simulink model "StampFly_StudentBlocks"  (R2026b)
settings: Solver=VariableStepAuto
undefined symbols (not defined in the file): Bottom, Official
(part 5 of 6)

== stateflow chart StampFly_StudentBlocks/Estimation/ToFHoldOutlierFilter ==
  note: ToF処理：新データ時に距離を更新。20 mm以下は保持、500 mmを超える飛びは最大2回補外。5 msフィルター。
  state Calculate
    en: [alt,raw]=stepFn(mm,fresh,mode,dt);
    du: [alt,raw]=stepFn(mm,fresh,mode,dt);
  (default) -> Calculate
  data: mm function_input; fresh function_input; mode function_input; dt function_input; alt function_output; raw function_output; mm input int16; fresh input uint8; mode input uint8; dt input single; alt output single; raw output int16
  function [alt,raw]=stepFn(mm,fresh,mode,dt):
    | function [alt,raw]=stepFn(mm,fresh,mode,dt)
    | % 日本語の説明はブロック注釈とDescriptionを参照。
    | %#codegen
    | persistent History Range Raw Outlier Alt PreviousMode;
    | if isempty(History)
    | History=zeros(4,1,'int16');
    | Range=int16(0);
    | Raw=int16(0);
    | Outlier=uint8(0);
    | Alt=single(0);
    | PreviousMode=uint8(0);
    | end
    |             if mode==3 && mode~=PreviousMode,History(:)=int16(0);Alt=single(0);end
    |             if mode>1
    |                 if fresh~=0
    |                     Raw=mm;if mm>int16(20),Range=mm;end
    |                     delta=int32(Range)-int32(History(2));
    |                     if abs(delta)>int32(500) && Outlier<uint8(2)
    |                         extrap=int32(History(2))+idivide(int32(History(2))-int32(History(4)),int32(2),'fix');
    |                         Range=int16(extrap);Outlier=Outlier+uint8(1);
    |                     else
    |                         Outlier=uint8(0);History(4)=History(3);History(3)=History(2);History(2)=Range;
    |                     end
    |                 end
    |                 Alt=filterStep(single(double(Range)/1000),dt,single(0.005),Alt);
    |             end
    |             alt=Alt;raw=Raw;PreviousMode=mode;
    | end
    | 
    | function s = filterStep(u,h,T,s)
    | %FILTERSTEP Exact Filter::update, including operation ordering.
    | %#codegen
    | s = s*T/(T+h) + u*h/(T+h);
    | end

== stateflow chart StampFly_StudentBlocks/LoggingAndStatus/StatusOutputs400/StatusIndicators400 ==
  note: LED・ブザー：校正、待機、飛行、低電圧、通信異常とモード変更を表示。色・周波数・再起動判定はモデル内。ハードウェアブロックは受け取った値だけを出力。
  state Calculate
    en: [color1,color2,tone,restart]=stepFn(mode,controlMode,altFlag,flipFlag,lowVoltage,rcError,ahrsFlag,button);
    du: [color1,color2,tone,restart]=stepFn(mode,controlMode,altFlag,flipFlag,lowVoltage,rcError,ahrsFlag,button);
  (default) -> Calculate
  data: arg_mode function_input; arg_controlMode function_input; arg_altFlag function_input; arg_flipFlag function_input; arg_lowVoltage function_input; arg_rcError function_input; arg_ahrsFlag function_input; arg_button function_input; arg_color1 function_output; arg_color2 function_output; arg_tone function_output; arg_restart function_output; mode input uint8; controlMode input single; altFlag input uint8; flipFlag input uint8; lowVoltage input uint8; rcError input uint8; ahrsFlag input uint8; button input uint8; color1 output uint32; color2 output uint32; tone output uint32; restart output boolean
  function [arg_color1,arg_color2,arg_tone,arg_restart]=stepFn(arg_mode,arg_controlMode,arg_altFlag,arg_flipFlag,arg_lowVoltage,arg_rcError,arg_ahrsFlag,arg_button):
    | function [arg_color1,arg_color2,arg_tone,arg_restart]=stepFn(arg_mode,arg_controlMode,arg_altFlag,arg_flipFlag,arg_lowVoltage,arg_rcError,arg_ahrsFlag,arg_button)
    | % 公式led_driveの状態色。ブザーの200ms待機は400Hzカウンターへ置換。
    | %#codegen
    | persistent Blink Rainbow C1 C2 Tick AHRSPrev ToneTicks ButtonCount WasPressed;
    | if isempty(Blink)
    |  Blink=uint16(0);Rainbow=uint32(255);C1=uint32(0);C2=uint32(0);Tick=uint16(0);AHRSPrev=uint8(0);ToneTicks=uint16(0);ButtonCount=uint8(0);WasPressed=false;
    | end
    | if arg_mode==1,C1=uint32(hex2dec('FF00FF'));C2=C1;
    | elseif arg_mode==5,C1=uint32(hex2dec('00FF00'));C2=C1;
    | elseif arg_mode==2
    |  c=uint32(hex2dec('FFFF00'));
    |  if arg_controlMode~=0,c=uint32(hex2dec('DC669B'));elseif arg_flipFlag~=0,c=uint32(hex2dec('FF9933'));end
    |  if arg_altFlag>=1,c=uint32(hex2dec('331155'));end
    |  if arg_rcError==1,c=uint32(hex2dec('FF0000'));end
    |  C1=c;C2=c;if arg_lowVoltage>=100,C1=uint32(hex2dec('18EBF9'));end
    | elseif arg_mode==3
    |  if arg_lowVoltage<100
    |   if Blink==0
    |    top=bitand(Rainbow,uint32(hex2dec('800000')))~=0;Rainbow=bitshift(Rainbow,1);if top,Rainbow=bitor(Rainbow,uint32(1));end
    |    C1=Rainbow;C2=Rainbow;Blink=Blink+uint16(1);
    |   end
    |   Blink=Blink+uint16(1);if Blink>20,Blink=uint16(0);end
    |  else
    |   if Blink<10,C1=uint32(hex2dec('18EBF9'));C2=C1;
    |   elseif Blink<200,C1=uint32(0);C2=uint32(0);else,Blink=uint16(0);end
    |   Blink=Blink+uint16(1);
    |  end
    |  if arg_ahrsFlag~=AHRSPrev && arg_ahrsFlag==1,ToneTicks=uint16(80);end
    |  AHRSPrev=arg_ahrsFlag;
    | end
    | arg_tone=uint32(0);
    | % Startup notes from official buzzer.h. Four 200ms notes, then silence.
    | if Tick<320
    |  notes=uint32([294 441 350 393]);idx=min(floor(double(Tick)/80)+1,4);arg_tone=notes(idx);Tick=Tick+uint16(1);
    | elseif ToneTicks>0,arg_tone=uint32(4000);ToneTicks=ToneTicks-uint16(1);end
    | arg_restart=false;
    | if arg_button==1,ButtonCount=min(ButtonCount+uint8(1),uint8(40));if ButtonCount>=4,WasPressed=true;end
    | elseif WasPressed,arg_restart=true;WasPressed=false;ButtonCount=uint8(0);else,ButtonCount=uint8(0);end
    | % FastLED brightness15, show32: cap displayed channels without changing logic.
    | arg_color1=scale(C1);arg_color2=scale(C2);
    | end
    | function c=scale(x)
    | r=bitand(bitshift(x,-16),uint32(255));g=bitand(bitshift(x,-8),uint32(255));b=bitand(x,uint32(255));
    | c=bitor(bitor(bitshift(uint32(double(r)*15/255),16),bitshift(uint32(double(g)*15/255),8)),uint32(double(b)*15/255));
    | end

== stateflow chart StampFly_StudentBlocks/Estimation/AltitudeKalman ==
  note: 高度Kalman：状態=[鉛直速度;高度;加速度バイアス]。400 Hzで最新保持ToFと鉛直加速度を使用。公式resetは内部推定xを保持。
  state Calculate
    en: [height,velocity,bias]=stepFn(alt,az,mode,dt,parkingReset);
    du: [height,velocity,bias]=stepFn(alt,az,mode,dt,parkingReset);
  (default) -> Calculate
  data: alt function_input; az function_input; mode function_input; dt function_input; parkingReset function_input; height function_output; velocity function_output; bias function_output; alt input single; az input single; mode input uint8; dt input single; parkingReset input boolean; height output single; velocity output single; bias output single
  function [height,velocity,bias]=stepFn(alt,az,mode,dt,parkingReset):
    | function [height,velocity,bias]=stepFn(alt,az,mode,dt,parkingReset)
    | % 日本語の説明はブロック注釈とDescriptionを参照。
    | %#codegen
    | persistent State First PreviousMode;
    | if isempty(State)
    | State=kalmanInitial();
    | First=false;
    | PreviousMode=uint8(0);
    | end
    |             if parkingReset,[~,State]=kalmanStep(single(0),single(0),dt,true,State);end
    |             if mode==3 && mode~=PreviousMode,First=false;end
    |             if mode>1
    |                 if First,[~,State]=kalmanStep(alt,az,dt,false,State);else,First=true;end
    |             end
    |             velocity=State.output(1);height=State.output(2);bias=State.output(3);PreviousMode=mode;
    | end
    | 
    | function [y,s] = kalmanStep(z,acc,h,resetState,s)
    | %KALMANSTEP Direct translation of Alt_kalman::update, state [v;z;bias].
    | % Preserve reset(): covariance and public output reset, private x is retained.
    | %#codegen
    | if resetState
    |     s.P = single(100)*eye(3,'single'); s.output(:) = single(0);
    | else
    |     p=s.P; b=single(-0.01); f=single(1)+h*b;
    |     xp=[s.x(1)+(acc-s.x(3))*h;s.x(2)+s.x(1)*h;s.x(3)*f];
    |     pp=zeros(3,3,'single');
    |     pp(1,1)=p(1,1)-h*(p(3,1)+p(1,3))+h*h*p(3,3)+h*h*single(0.01);
    |     pp(1,2)=h*(p(1,1)-p(3,2))-h*h*p(3,1)+p(1,2);
    |     pp(1,3)=f*(p(1,3)-h*p(3,3));
    |     pp(2,1)=h*(p(1,1)-p(2,3))-h*h*p(1,3)+p(2,1);
    |     pp(2,2)=h*h*p(1,1)+h*(p(2,1)+p(1,2))+p(2,2);
    |     pp(2,3)=f*(p(2,3)+h*p(1,3));
    |     pp(3,1)=f*(p(3,1)-h*p(3,3));
    |     pp(3,2)=f*(p(3,2)+h*p(3,1));
    |     pp(3,3)=f*f*p(3,3)+h*h;
    |     k=[pp(1,2);pp(2,2);pp(3,2)]/(pp(2,2)+single(0.004*0.004));
    |     e=z-xp(2); s.x=xp+k*e; s.output=s.x;
    |     s.P(1,:)=pp(1,:)-k(1)*pp(2,:);
    |     s.P(2,:)=pp(2,:)*(single(1)-k(2));
    |     s.P(3,:)=-k(3)*pp(2,:)+pp(3,:);
    | end
    | y=s.output;
    | end
    | 
    | function s = kalmanInitial()
    | %#codegen
    | s = struct('x',zeros(3,1,'single'),'P',single(100)*eye(3,'single'), ...
    |     'output',zeros(3,1,'single'));
    | end

== stateflow chart StampFly_StudentBlocks/Estimation/SensorFlags ==
  note: フラグ判定：OverG、距離無効/高度上限、低電圧100回。PID制御や状態遷移で使います。
  state Calculate
    en: [flags]=stepFn(accel,azd,voltage,mode,altFlag,height,rawRange,dt,parkingReset,flipFlag);
    du: [flags]=stepFn(accel,azd,voltage,mode,altFlag,height,rawRange,dt,parkingReset,flipFlag);
  (default) -> Calculate
  data: arg_accel function_input; arg_azd function_input; arg_voltage function_input; arg_mode function_input; arg_altFlag function_input; arg_height function_input; arg_rawRange function_input; arg_dt function_input; arg_parkingReset function_input; arg_flags function_output; arg_flipFlag function_input; accel input single; azd input single; voltage input single; mode input uint8; altFlag input uint8; height input single; rawRange input int16; dt input single; parkingReset input boolean; flags output uint8; flipFlag input uint8
  function arg_flags =stepFn(arg_accel,arg_azd,arg_voltage,arg_mode,arg_altFlag,arg_height,arg_rawRange,arg_dt,arg_parkingReset,arg_flipFlag):
    | function arg_flags =stepFn(arg_accel,arg_azd,arg_voltage,arg_mode,arg_altFlag,arg_height,arg_rawRange,arg_dt,arg_parkingReset,arg_flipFlag)
    | % 日本語の説明はブロック注釈とDescriptionを参照。
    | %#codegen
    | persistent Norm Voltage OverG RangeFlag LowVoltage PreviousMode;
    | if isempty(Norm)
    | Norm=single(0);
    | Voltage=single(0);
    | OverG=uint8(0);
    | RangeFlag=uint8(0);
    | LowVoltage=uint8(0);
    | PreviousMode=uint8(0);
    | end
    |             if arg_parkingReset,OverG=uint8(0);RangeFlag=uint8(0);end
    |             if arg_mode==3 && arg_mode~=PreviousMode,Norm=single(0);end
    |             if arg_mode>1
    |                 if (arg_height>single(2) && arg_altFlag~=0 && arg_flipFlag==0) || arg_rawRange==0,RangeFlag=min(RangeFlag+uint8(1),uint8(20));else,RangeFlag=uint8(0);end
    |             end
    |             normA=sqrt(arg_accel(1)*arg_accel(1)+arg_accel(2)*arg_accel(2)+arg_azd*arg_azd);
    |             Norm=filterStep(normA,arg_dt,single(.005),Norm);
    |             if Norm>single(2),OverG=uint8(1);end
    |             Voltage=filterStep(arg_voltage,arg_dt,single(.005),Voltage);
    |             if LowVoltage~=uint8(100)
    |                 if Voltage<single(3.34),LowVoltage=LowVoltage+uint8(1);else,LowVoltage=uint8(0);end
    |                 LowVoltage=min(LowVoltage,uint8(100));
    |             end
    |             arg_flags=[OverG;RangeFlag;LowVoltage];PreviousMode=arg_mode;
    | end
    | 
    | function s = filterStep(u,h,T,s)
    | %FILTERSTEP Exact Filter::update, including operation ordering.
    | %#codegen
    | s = s*T/(T+h) + u*h/(T+h);
    | end

== stateflow chart StampFly_StudentBlocks/Estimation/SensorProcessing400/AltitudeKalman ==
  note: 高度Kalman：状態=[鉛直速度;高度;加速度バイアス]。400 Hzで最新保持ToFと鉛直加速度を使用。公式resetは内部推定xを保持。
  state Calculate
    en: [height,velocity,bias]=stepFn(alt,az,mode,dt,parkingReset);
    du: [height,velocity,bias]=stepFn(alt,az,mode,dt,parkingReset);
  (default) -> Calculate
  data: alt function_input; az function_input; mode function_input; dt function_input; parkingReset function_input; height function_output; velocity function_output; bias function_output; alt input single; az input single; mode input uint8; dt input single; parkingReset input boolean; height output single; velocity output single; bias output single
  function [height,velocity,bias]=stepFn(alt,az,mode,dt,parkingReset):
    | function [height,velocity,bias]=stepFn(alt,az,mode,dt,parkingReset)
    | % 日本語の説明はブロック注釈とDescriptionを参照。
    | %#codegen
    | persistent State First PreviousMode;
    | if isempty(State)
    | State=kalmanInitial();
    | First=false;
    | PreviousMode=uint8(0);
    | end
    |             if parkingReset,[~,State]=kalmanStep(single(0),single(0),dt,true,State);end
    |             if mode==3 && mode~=PreviousMode,First=false;end
    |             if mode>1
    |                 if First,[~,State]=kalmanStep(alt,az,dt,false,State);else,First=true;end
    |             end
    |             velocity=State.output(1);height=State.output(2);bias=State.output(3);PreviousMode=mode;
    | end
    | 
    | function [y,s] = kalmanStep(z,acc,h,resetState,s)
    | %KALMANSTEP Direct translation of Alt_kalman::update, state [v;z;bias].
    | % Preserve reset(): covariance and public output reset, private x is retained.
    | %#codegen
    | if resetState
    |     s.P = single(100)*eye(3,'single'); s.output(:) = single(0);
    | else
    |     p=s.P; b=single(-0.01); f=single(1)+h*b;
    |     xp=[s.x(1)+(acc-s.x(3))*h;s.x(2)+s.x(1)*h;s.x(3)*f];
    |     pp=zeros(3,3,'single');
    |     pp(1,1)=p(1,1)-h*(p(3,1)+p(1,3))+h*h*p(3,3)+h*h*single(0.01);
    |     pp(1,2)=h*(p(1,1)-p(3,2))-h*h*p(3,1)+p(1,2);
    |     pp(1,3)=f*(p(1,3)-h*p(3,3));
    |     pp(2,1)=h*(p(1,1)-p(2,3))-h*h*p(1,3)+p(2,1);
    |     pp(2,2)=h*h*p(1,1)+h*(p(2,1)+p(1,2))+p(2,2);
    |     pp(2,3)=f*(p(2,3)+h*p(1,3));
    |     pp(3,1)=f*(p(3,1)-h*p(3,3));
    |     pp(3,2)=f*(p(3,2)+h*p(3,1));
    |     pp(3,3)=f*f*p(3,3)+h*h;
    |     k=[pp(1,2);pp(2,2);pp(3,2)]/(pp(2,2)+single(0.004*0.004));
    |     e=z-xp(2); s.x=xp+k*e; s.output=s.x;
    |     s.P(1,:)=pp(1,:)-k(1)*pp(2,:);
    |     s.P(2,:)=pp(2,:)*(single(1)-k(2));
    |     s.P(3,:)=-k(3)*pp(2,:)+pp(3,:);
    | end
    | y=s.output;
    | end
    | 
    | function s = kalmanInitial()
    | %#codegen
    | s = struct('x',zeros(3,1,'single'),'P',single(100)*eye(3,'single'), ...
    |     'output',zeros(3,1,'single'));
    | end

== stateflow chart StampFly_StudentBlocks/Estimation/SensorProcessing400/IMUAxisConversion ==
  note: IMU軸変換：センサーX/Yを入れ替えZの符号を反転。公式の加速度単位gを保持します。
  state Calculate
    en: [a,g]=stepFn(accelMps2,gyroRps);
    du: [a,g]=stepFn(accelMps2,gyroRps);
  (default) -> Calculate
  data: accelMps2 function_input; gyroRps function_input; a function_output; g function_output; accelMps2 input single; gyroRps input single; a output single; g output single
  function [a,g]=stepFn(accelMps2,gyroRps):
    | function [a,g]=stepFn(accelMps2,gyroRps)
    | % 日本語の説明はブロック注釈とDescriptionを参照。
    | %#codegen
    |             a=accelMps2([2 1 3])/single(9.80665);a(3)=-a(3);
    |             g=gyroRps([2 1 3]);g(3)=-g(3);
    | end

== stateflow chart StampFly_StudentBlocks/Estimation/SensorProcessing400/IMUBiasCalibration ==
  note: 800周期の平均校正：ジャイロXYZと加速度Zのオフセットを平均します。400 Hzなので公称2秒です。
  state Calculate
    en: [offset,count]=stepFn(a,g,mode);
    du: [offset,count]=stepFn(a,g,mode);
  (default) -> Calculate
  data: a function_input; g function_input; mode function_input; offset function_output; count function_output; a input single; g input single; mode input uint8; offset output single; count output uint16
  function [offset,count]=stepFn(a,g,mode):
    | function [offset,count]=stepFn(a,g,mode)
    | % 日本語の説明はブロック注釈とDescriptionを参照。
    | %#codegen
    | persistent Offset Count;
    | if isempty(Offset)
    | Offset=zeros(4,1,'single');
    | Count=uint16(0);
    | end
    |             if mode==0,Offset(:)=single(0);Count=uint16(0);
    |             elseif mode==1 && Count<uint16(800)
    |                 n=single(Count);Offset=(n*Offset+[g;a(3)])/(n+single(1));Count=Count+uint16(1);
    |             end
    |             offset=Offset;count=Count;
    | end

== stateflow chart StampFly_StudentBlocks/Estimation/SensorProcessing400/IMUFiltering ==
  note: IMUフィルター：加速度とジャイロは時定数3 ms、鉛直差分は100 ms。PARKING移行で状態をリセット。
  state Calculate
    en: [af,gf,azd]=stepFn(a,g,offset,mode,dt);
    du: [af,gf,azd]=stepFn(a,g,offset,mode,dt);
  (default) -> Calculate
  data: a function_input; g function_input; offset function_input; mode function_input; dt function_input; af function_output; gf function_output; azd function_output; a input single; g input single; offset input single; mode input uint8; dt input single; af output single; gf output single; azd output single
  function [af,gf,azd]=stepFn(a,g,offset,mode,dt):
    | function [af,gf,azd]=stepFn(a,g,offset,mode,dt)
    | % 日本語の説明はブロック注釈とDescriptionを参照。
    | %#codegen
    | persistent Filter Accel Gyro Azd PreviousMode;
    | if isempty(Filter)
    | Filter=zeros(7,1,'single');
    | Accel=zeros(3,1,'single');
    | Gyro=zeros(3,1,'single');
    | Azd=single(0);
    | PreviousMode=uint8(0);
    | end
    |             if mode==3 && mode~=PreviousMode,Filter(:)=single(0);end
    |             if mode>1
    |                 for j=1:3
    |                     Filter(j)=filterStep(a(j),dt,single(0.003),Filter(j));
    |                     Filter(j+3)=filterStep(g(j)-offset(j),dt,single(0.003),Filter(j+3));
    |                 end
    |                 Filter(7)=filterStep(a(3)-offset(4),dt,single(0.1),Filter(7));
    |                 Accel=Filter(1:3);Gyro=Filter(4:6);Azd=Filter(7);
    |             end
    |             af=Accel;gf=Gyro;azd=Azd;PreviousMode=mode;
    | end
    | 
    | function s = filterStep(u,h,T,s)
    | %FILTERSTEP Exact Filter::update, including operation ordering.
    | %#codegen
    | s = s*T/(T+h) + u*h/(T+h);
    | end

== stateflow chart StampFly_StudentBlocks/Estimation/SensorProcessing400/MadgwickAttitude ==
  note: Madgwick姿勢推定：400 Hz、β=0.1。公式の高速逆平方根、軸の対応、Yaw+180°を保持。数式はこのChart内にあります。
  state Calculate
    en: [a,q]=stepFn(rates,accel,mode,reset);
    du: [a,q]=stepFn(rates,accel,mode,reset);
  (default) -> Calculate
  data: arg_rates function_input; arg_accel function_input; arg_mode function_input; arg_reset function_input; arg_a function_output; arg_q function_output; rates input single; accel input single; mode input uint8; reset input boolean; a output single; q output single
  function [arg_a,arg_q]=stepFn(arg_rates,arg_accel,arg_mode,arg_reset):
    | function [arg_a,arg_q]=stepFn(arg_rates,arg_accel,arg_mode,arg_reset)
    | % 日本語の説明はブロック注釈とDescriptionを参照。
    | %#codegen
    | persistent Q Angles;
    | if isempty(Q)
    | Q=single([1;0;0;0]);
    | Angles=zeros(3,1,'single');
    | end
    |             if arg_reset,Q=single([1;0;0;0]);end
    |             if arg_mode>1,[Angles,Q]=madgwickStep(arg_rates,arg_accel,Q,false);end
    |             arg_a=Angles;arg_q=Q;
    | end
    | 
    | function [attitude,arg_q] = madgwickStep(arg_rates,arg_accel,arg_q,arg_reset)
    | %MADGWICKSTEP Official updateIMU with body-axis conventions and invSqrt.
    | % Rates rad/s and arg_accel g in official body frame [forward;left;down].
    | % Madgwick is fixed 400 Hz even though other official filters use measured dt.
    | % Translation of lib/MdgwickAHRS/MadgwickAHRS.cpp; original license retained.
    | %#codegen
    | if arg_reset, arg_q=single([1;0;0;0]); end
    | q0=arg_q(1);q1=arg_q(2);q2=arg_q(3);q3=arg_q(4);
    | % Retain original rad->deg->rad conversion coefficients, including rounding.
    | g=arg_rates([2 1 3])*single(180/pi);g(3)=-g(3);
    | g=g*single(0.0174533);gx=g(1);gy=g(2);gz=g(3);
    | arg_a=arg_accel([2 1 3]);arg_a(3)=-arg_a(3);ax=arg_a(1);ay=arg_a(2);az=arg_a(3);
    | dq=single(0.5)*[-q1*gx-q2*gy-q3*gz; q0*gx+q2*gz-q3*gy; ...
    |     q0*gy-q1*gz+q3*gx; q0*gz+q1*gy-q2*gx];
    | if ax~=0 || ay~=0 || az~=0
    |     reciprocal=fastInvSqrt(ax*ax+ay*ay+az*az);
    |     ax=ax*reciprocal;ay=ay*reciprocal;az=az*reciprocal;
    |     q02=q0*q0;q12=q1*q1;q22=q2*q2;q32=q3*q3;
    |     q0x2=single(2)*q0;q1x2=single(2)*q1;q2x2=single(2)*q2;q3x2=single(2)*q3;
    |     q0x4=single(4)*q0;q1x4=single(4)*q1;q2x4=single(4)*q2;
    |     q1x8=single(8)*q1;q2x8=single(8)*q2;
    |     gradient=[q0x4*q22+q2x2*ax+q0x4*q12-q1x2*ay; ...
    |         q1x4*q32-q3x2*ax+single(4)*q02*q1-q0x2*ay-q1x4+q1x8*q12+q1x8*q22+q1x4*az; ...
    |         single(4)*q02*q2+q0x2*ax+q2x4*q32-q3x2*ay-q2x4+q2x8*q12+q2x8*q22+q2x4*az; ...
    |         single(4)*q12*q3-q1x2*ax+single(4)*q22*q3-q2x2*ay];
    |     reciprocal=fastInvSqrt(gradient(1)*gradient(1)+gradient(2)*gradient(2)+gradient(3)*gradient(3)+gradient(4)*gradient(4));
    |     gradient=gradient*reciprocal;
    |     dq=dq-single(0.1)*gradient;
    | end
    | arg_q=arg_q+dq*single(1/400);
    | reciprocal=fastInvSqrt(arg_q(1)*arg_q(1)+arg_q(2)*arg_q(2)+arg_q(3)*arg_q(3)+arg_q(4)*arg_q(4));arg_q=arg_q*reciprocal;
    | roll=atan2(arg_q(1)*arg_q(2)+arg_q(3)*arg_q(4),single(0.5)-arg_q(2)*arg_q(2)-arg_q(3)*arg_q(3));
    | pitch=asin(-single(2)*(arg_q(2)*arg_q(4)-arg_q(1)*arg_q(3)));
    | yaw=atan2(arg_q(2)*arg_q(3)+arg_q(1)*arg_q(4),single(0.5)-arg_q(3)*arg_q(3)-arg_q(4)*arg_q(4));
    | % Original getYaw adds 180 degrees; do not hide this offset.
    | attitude=[pitch*single(57.29578);roll*single(57.29578); ...
    |     -(yaw*single(57.29578)+single(180))]*single(pi/180);
    | end
    | 
    | function y=fastInvSqrt(x)
    | i=typecast(x,'uint32');i=uint32(hex2dec('5f3759df'))-bitshift(i,-1);
    | y=typecast(i,'single');half=single(0.5)*x;
    | y=y*(single(1.5)-half*y*y);y=y*(single(1.5)-half*y*y);
    | end

== stateflow chart StampFly_StudentBlocks/Estimation/SensorProcessing400/SensorDiagnosticPack ==
  state Calculate
    en: [diag]=stepFn(az,bias,alt,offset,count);
    du: [diag]=stepFn(az,bias,alt,offset,count);
  (default) -> Calculate
  data: az function_input; bias function_input; alt function_input; offset function_input; count function_input; diag function_output; az input single; bias input single; alt input single; offset input single; count input uint16; diag output single
  function diag =stepFn(az,bias,alt,offset,count):
    | function diag =stepFn(az,bias,alt,offset,count)
    | % 日本語の説明はブロック注釈とDescriptionを参照。
    | %#codegen
    |             diag=[az;bias;alt;offset;single(count)];
    | end

== stateflow chart StampFly_StudentBlocks/Estimation/SensorProcessing400/SensorFlags ==
  note: フラグ判定：OverG、距離無効/高度上限、低電圧100回。PID制御や状態遷移で使います。
  state Calculate
    en: [flags]=stepFn(accel,azd,voltage,mode,altFlag,height,rawRange,dt,parkingReset,flipFlag);
    du: [flags]=stepFn(accel,azd,voltage,mode,altFlag,height,rawRange,dt,parkingReset,flipFlag);
  (default) -> Calculate
  data: arg_accel function_input; arg_azd function_input; arg_voltage function_input; arg_mode function_input; arg_altFlag function_input; arg_height function_input; arg_rawRange function_input; arg_dt function_input; arg_parkingReset function_input; arg_flags function_output; arg_flipFlag function_input; accel input single; azd input single; voltage input single; mode input uint8; altFlag input uint8; height input single; rawRange input int16; dt input single; parkingReset input boolean; flags output uint8; flipFlag input uint8
  function arg_flags =stepFn(arg_accel,arg_azd,arg_voltage,arg_mode,arg_altFlag,arg_height,arg_rawRange,arg_dt,arg_parkingReset,arg_flipFlag):
    | function arg_flags =stepFn(arg_accel,arg_azd,arg_voltage,arg_mode,arg_altFlag,arg_height,arg_rawRange,arg_dt,arg_parkingReset,arg_flipFlag)
    | % 日本語の説明はブロック注釈とDescriptionを参照。
    | %#codegen
    | persistent Norm Voltage OverG RangeFlag LowVoltage PreviousMode;
    | if isempty(Norm)
    | Norm=single(0);
    | Voltage=single(0);
    | OverG=uint8(0);
    | RangeFlag=uint8(0);
    | LowVoltage=uint8(0);
    | PreviousMode=uint8(0);
    | end
    |             if arg_parkingReset,OverG=uint8(0);RangeFlag=uint8(0);end
    |             if arg_mode==3 && arg_mode~=PreviousMode,Norm=single(0);end
    |             if arg_mode>1
    |                 if (arg_height>single(2) && arg_altFlag~=0 && arg_flipFlag==0) || arg_rawRange==0,RangeFlag=min(RangeFlag+uint8(1),uint8(20));else,RangeFlag=uint8(0);end
    |             end
    |             normA=sqrt(arg_accel(1)*arg_accel(1)+arg_accel(2)*arg_accel(2)+arg_azd*arg_azd);
    |             Norm=filterStep(normA,arg_dt,single(.005),Norm);
    |             if Norm>single(2),OverG=uint8(1);end
    |             Voltage=filterStep(arg_voltage,arg_dt,single(.005),Voltage);
    |             if LowVoltage~=uint8(100)
    |                 if Voltage<single(3.34),LowVoltage=LowVoltage+uint8(1);else,LowVoltage=uint8(0);end
    |                 LowVoltage=min(LowVoltage,uint8(100));
    |             end
    |             arg_flags=[OverG;RangeFlag;LowVoltage];PreviousMode=arg_mode;
    | end
    | 
    | function s = filterStep(u,h,T,s)
    | %FILTERSTEP Exact Filter::update, including operation ordering.
    | %#codegen
    | s = s*T/(T+h) + u*h/(T+h);
    | end

== stateflow chart StampFly_StudentBlocks/Estimation/SensorProcessing400/ToFHoldOutlierFilter ==
  note: ToF処理：新データ時に距離を更新。20 mm以下は保持、500 mmを超える飛びは最大2回補外。5 msフィルター。
  state Calculate
    en: [alt,raw]=stepFn(mm,fresh,mode,dt);
    du: [alt,raw]=stepFn(mm,fresh,mode,dt);
  (default) -> Calculate
  data: mm function_input; fresh function_input; mode function_input; dt function_input; alt function_output; raw function_output; mm input int16; fresh input uint8; mode input uint8; dt input single; alt output single; raw output int16
  function [alt,raw]=stepFn(mm,fresh,mode,dt):
    | function [alt,raw]=stepFn(mm,fresh,mode,dt)
    | % 日本語の説明はブロック注釈とDescriptionを参照。
    | %#codegen
    | persistent History Range Raw Outlier Alt PreviousMode;
    | if isempty(History)
    | History=zeros(4,1,'int16');
    | Range=int16(0);
    | Raw=int16(0);
    | Outlier=uint8(0);
    | Alt=single(0);
    | PreviousMode=uint8(0);
    | end
    |             if mode==3 && mode~=PreviousMode,History(:)=int16(0);Alt=single(0);end
    |             if mode>1
    |                 if fresh~=0
    |                     Raw=mm;if mm>int16(20),Range=mm;end
    |                     delta=int32(Range)-int32(History(2));
    |                     if abs(delta)>int32(500) && Outlier<uint8(2)
    |                         extrap=int32(History(2))+idivide(int32(History(2))-int32(History(4)),int32(2),'fix');
    |                         Range=int16(extrap);Outlier=Outlier+uint8(1);
    |                     else
    |                         Outlier=uint8(0);History(4)=History(3);History(3)=History(2);History(2)=Range;
    |                     end
    |                 end
    |                 Alt=filterStep(single(double(Range)/1000),dt,single(0.005),Alt);
    |             end
    |             alt=Alt;raw=Raw;PreviousMode=mode;
    | end
    | 
    | function s = filterStep(u,h,T,s)
    | %FILTERSTEP Exact Filter::update, including operation ordering.
    | %#codegen
    | s = s*T/(T+h) + u*h/(T+h);
    | end

== stateflow chart StampFly_StudentBlocks/Estimation/SensorProcessing400/VerticalAcceleration ==
  note: 鉛直加速度：校正後AccelZ差分を反転して100 msフィルター。公式に合わせ単位gのまま高度Kalmanへ入力。
  state Calculate
    en: [az]=stepFn(azd,mode,dt);
    du: [az]=stepFn(azd,mode,dt);
  (default) -> Calculate
  data: azd function_input; mode function_input; dt function_input; az function_output; azd input single; mode input uint8; dt input single; az output single
  function az =stepFn(azd,mode,dt):
    | function az =stepFn(azd,mode,dt)
    | % 日本語の説明はブロック注釈とDescriptionを参照。
    | %#codegen
    | persistent Az PreviousMode;
    | if isempty(Az)
    | Az=single(0);
    | PreviousMode=uint8(0);
    | end
    |             if mode==3 && mode~=PreviousMode,Az=single(0);end
    |             if mode>1,Az=filterStep(-azd,dt,single(0.1),Az);end
    |             az=Az;PreviousMode=mode;
    | end
    | 
    | function s = filterStep(u,h,T,s)
    | %FILTERSTEP Exact Filter::update, including operation ordering.
    | %#codegen
    | s = s*T/(T+h) + u*h/(T+h);
    | end

== stateflow chart StampFly_StudentBlocks/FlightSequence/OfficialFlightSupervisor ==
  note: 公式の状態監督：INIT=0 → AVERAGE=1 → PARKING=3 → FLIGHT=2。ボタン・通信喪失・センサー状態に応じて LANDING=5 へ遷移。押下・解放の判定順を公式と一致させる。
  state Calculate
    en: [branch,mode,ahrsReset,parkingReset,connected]=stepFn(previousMode,button,newPacket,flags,ahrsFlag);
    du: [branch,mode,ahrsReset,parkingReset,connected]=stepFn(previousMode,button,newPacket,flags,ahrsFlag);
  (default) -> Calculate
  data: arg_previousMode function_input; arg_button function_input; arg_newPacket function_input; arg_flags function_input; arg_ahrsFlag function_input; arg_branch function_output; arg_mode function_output; arg_ahrsReset function_output; arg_parkingReset function_output; arg_connected function_output; previousMode input uint8; button input uint8; newPacket input uint8; flags input uint8; ahrsFlag input uint8; branch output uint8; mode output uint8; ahrsReset output boolean; parkingReset output boolean; connected output uint8
  function [arg_branch,arg_mode,arg_ahrsReset,arg_parkingReset,arg_connected]=stepFn(arg_previousMode,arg_button,arg_newPacket,arg_flags,arg_ahrsFlag):
    | function [arg_branch,arg_mode,arg_ahrsReset,arg_parkingReset,arg_connected]=stepFn(arg_previousMode,arg_button,arg_newPacket,arg_flags,arg_ahrsFlag)
    | % 公式loop_400Hzの分岐開始時。遷移後も現在の分岐を最後まで実行する。
    | %#codegen
    | persistent calibration buttonCounter buttonState chatter lastAHRS connectionCounter;
    | if isempty(calibration)
    |  calibration=uint16(0);buttonCounter=int8(0);buttonState=uint8(0);
    |  chatter=uint8(0);lastAHRS=uint8(0);connectionCounter=uint16(0);
    | end
    | arg_branch=arg_previousMode;arg_mode=arg_branch;arg_ahrsReset=false;arg_parkingReset=arg_branch==3;
    | if arg_newPacket~=0,connectionCounter=uint16(0);end
    | arg_connected=uint8(connectionCounter<uint16(40));
    | if arg_branch==0,arg_mode=uint8(1);
    | elseif arg_branch==1
    |  if calibration<uint16(800),calibration=calibration+uint16(1);else,arg_mode=uint8(3);end
    | else
    |  if arg_button==1
    |   buttonCounter=buttonCounter+int8(1);
    |   if buttonCounter>int8(10),buttonCounter=int8(10);buttonState=uint8(1);end
    |  else
    |   buttonCounter=buttonCounter-int8(1);
    |   if buttonCounter<int8(-10),buttonCounter=int8(-10);buttonState=uint8(0);end
    |  end
    |  event=false;
    |  if chatter==0
    |   if buttonState==1,chatter=uint8(1);end
    |  elseif buttonState==0
    |   chatter=chatter+uint8(1);
    |   if chatter>uint8(40),chatter=uint8(0);event=true;end
    |  end
    |  if arg_branch==3
    |   if event,arg_mode=uint8(2);arg_ahrsReset=true;end
    |   if arg_ahrsFlag~=lastAHRS
    |    if arg_ahrsFlag==1,arg_ahrsReset=true;end
    |    lastAHRS=arg_ahrsFlag;
    |   end
    |  elseif arg_branch==2 || arg_branch==6
    |   connectionCounter=uint16(mod(double(connectionCounter)+1,65536));
    |   arg_connected=uint8(connectionCounter<uint16(40));
    |   if event,arg_mode=uint8(5);end
    |   if arg_connected==0,arg_mode=uint8(5);end
    |   if arg_flags(1)==1,arg_mode=uint8(3);end
    |   if arg_branch==2 && arg_mode~=arg_branch,arg_ahrsReset=true;end
    |  elseif arg_branch==5
    |   if event,arg_mode=uint8(3);end
    |  end
    | end
    | end

== stateflow chart StampFly_StudentBlocks/FlightSequence/OfficialFlipSequence ==
  note: 公式 Flip：ボタンで開始し、推力・Roll角速度を段階的に切り替える。完了・中断時の保持値と推定器のリセットを公式の順に出力。USBベンチでは実モーター出力ゼロ。
  state Calculate
    en: [start,done,phase,thrust,rollRate,angleReset,ahrsReset,normalControl]=stepFn(button,branch,voltage,previousReset,lastRate);
    du: [start,done,phase,thrust,rollRate,angleReset,ahrsReset,normalControl]=stepFn(button,branch,voltage,previousReset,lastRate);
  (default) -> Calculate
  data: arg_arg_button function_input; arg_arg_branch function_input; arg_arg_voltage function_input; arg_arg_previousReset function_input; arg_arg_lastRate function_input; arg_arg_start function_output; arg_arg_done function_output; arg_arg_phase function_output; arg_arg_thrust function_output; arg_arg_rollRate function_output; arg_arg_angleReset function_output; arg_arg_ahrsReset function_output; arg_arg_normalControl function_output; button input uint8; branch input uint8; voltage input single; previousReset input boolean; lastRate input single; start output boolean; done output boolean; phase output uint8; thrust output single; rollRate output single; angleReset output boolean; ahrsReset output boolean; normalControl output boolean
  function [arg_arg_start,arg_arg_done,arg_arg_phase,arg_arg_thrust,arg_arg_rollRate,arg_arg_angleReset,arg_arg_ahrsReset,arg_arg_normalControl]=stepFn(arg_arg_button,arg_arg_branch,arg_arg_voltage,arg_arg_previousReset,arg_arg_lastRate):
    | function [arg_arg_start,arg_arg_done,arg_arg_phase,arg_arg_thrust,arg_arg_rollRate,arg_arg_angleReset,arg_arg_ahrsReset,arg_arg_normalControl]=stepFn(arg_arg_button,arg_arg_branch,arg_arg_voltage,arg_arg_previousReset,arg_arg_lastRate)
    | % 公式 flip(): 180 + 40*4 + 10 + 190 tick。制御は別のPIDブロック。
    | %#codegen
    | persistent counter buttonCount rate didReset;
    | if isempty(counter),counter=uint16(0);buttonCount=uint8(0);rate=single(0);didReset=false;end
    | arg_arg_start=false;arg_arg_done=false;arg_arg_phase=uint8(0);arg_arg_thrust=single(0);arg_arg_rollRate=single(0);arg_arg_angleReset=false;arg_arg_ahrsReset=false;arg_arg_normalControl=true;
    | if arg_arg_branch==3 || arg_arg_previousReset,counter=uint16(0);rate=single(0);didReset=false;end
    | if arg_arg_branch==6
    |  rate=arg_arg_lastRate(1);
    |  T=single(double(-single(.2448)*arg_arg_voltage+single(1.5892))*3.7);
    |  flipTime=single(.4);flipStep=uint16(fix(flipTime/single(.0025)));quarter=idivide(flipStep,uint16(4));
    |  domega=single(double(single(.00217))*8*pi/double(flipTime)/double(flipTime));
    |  if counter<180
    |   arg_arg_phase=uint8(1);arg_arg_normalControl=false;
    |   if arg_arg_voltage>3.8,arg_arg_thrust=single(double(T)+.17*3.7);else,arg_arg_thrust=single(double(T)+.15*3.7);end
    |  elseif counter<180+quarter
    |   arg_arg_phase=uint8(2);arg_arg_normalControl=false;arg_arg_thrust=T*single(.3);rate=rate+domega;
    |  elseif counter<180+2*quarter
    |   arg_arg_phase=uint8(3);arg_arg_normalControl=false;arg_arg_thrust=T*single(.15);rate=rate+domega;
    |  elseif counter<180+3*quarter
    |   arg_arg_phase=uint8(4);arg_arg_normalControl=false;arg_arg_thrust=T*single(.15);rate=rate-domega;
    |  elseif counter<180+flipStep
    |   arg_arg_phase=uint8(5);arg_arg_normalControl=false;arg_arg_thrust=T;rate=rate-domega;
    |  elseif counter<190+flipStep
    |   arg_arg_phase=uint8(6);arg_arg_normalControl=false;arg_arg_thrust=single(double(T)+double(single(.18))*3.7);rate=single(0);arg_arg_angleReset=true;
    |   if ~didReset,arg_arg_ahrsReset=true;didReset=true;end
    |  elseif counter<380+flipStep,arg_arg_normalControl=true;
    |  else,arg_arg_done=true;arg_arg_normalControl=false;counter=uint16(0);didReset=false;
    |  end
    |  arg_arg_rollRate=rate;if ~arg_arg_done,counter=counter+uint16(1);end
    | end
    | if arg_arg_branch==2 || (arg_arg_branch==6 && arg_arg_normalControl)
    |  if arg_arg_button==1
    |   buttonCount=buttonCount+uint8(1);
    |   if buttonCount>uint8(10),buttonCount=uint8(0);arg_arg_start=true;end
    |  else,buttonCount=uint8(0);end
    | end
    | end

== stateflow chart StampFly_StudentBlocks/FlightSequence/TakeoffLandingCommand ==
  note: 離陸/着陸の指令：離陸カウンター0〜1000、初期高度0.5 m、上下スティックで0.05〜1.8 m。電圧トリム=-0.2448V+1.5892。
  state Calculate
    en: [alt,base,counter,raw,auto,manual,controlMode]=stepFn(stick,height,voltage,rangeFlag,mode,phase,flipDone);
    du: [alt,base,counter,raw,auto,manual,controlMode]=stepFn(stick,height,voltage,rangeFlag,mode,phase,flipDone);
  (default) -> Calculate
  data: arg_arg_stick function_input; arg_arg_height function_input; arg_arg_voltage function_input; arg_arg_rangeFlag function_input; arg_branch function_input; arg_arg_alt function_output; arg_arg_base function_output; arg_arg_counter function_output; arg_arg_raw function_output; arg_arg_auto function_output; arg_arg_manual function_output; arg_arg_phase function_input; arg_arg_flipDone function_input; arg_arg_controlMode function_output; stick input single; height input single; voltage input single; rangeFlag input uint8; mode input uint8; alt output single; base output single; counter output uint16; raw output single; auto output boolean; manual output boolean; phase input uint8; flipDone input boolean; controlMode output single
  function [arg_arg_alt,arg_arg_base,arg_arg_counter,arg_arg_raw,arg_arg_auto,arg_arg_manual,arg_arg_controlMode]=stepFn(arg_arg_stick,arg_arg_height,arg_arg_voltage,arg_arg_rangeFlag,arg_branch,arg_arg_phase,arg_arg_flipDone):
    | function [arg_arg_alt,arg_arg_base,arg_arg_counter,arg_arg_raw,arg_arg_auto,arg_arg_manual,arg_arg_controlMode]=stepFn(arg_arg_stick,arg_arg_height,arg_arg_voltage,arg_arg_rangeFlag,arg_branch,arg_arg_phase,arg_arg_flipDone)
    | % 公式get_command/auto_landing。Alt_flagはManual切替時にも保持される。
    | %#codegen
    | persistent Alt Base Counter RangeOld Landing History AltFlag ControlMode;
    | if isempty(Alt)
    |  Alt=single(.5);Base=single(0);Counter=uint16(0);RangeOld=uint8(0);
    |  Landing=false;History=zeros(10,1,'single');AltFlag=false;ControlMode=uint8(0);
    | end
    | arg_arg_raw=single(0);arg_arg_manual=false;
    | if arg_branch==3
    |  Base=single(0);Alt=single(.5);Counter=uint16(0);Landing=false;AltFlag=false;
    | elseif arg_branch==2 || (arg_branch==6 && arg_arg_phase==0 && ~arg_arg_flipDone)
    |  ControlMode=uint8(arg_arg_stick(5));
    |  if uint8(arg_arg_stick(6))==4
    |   AltFlag=true;
    |   if Counter<500
    |    Base=min(single(Counter)/single(1000),trim(single(3.8)));Counter=Counter+uint16(1);
    |   elseif Counter<1000
    |    Base=min(single(Counter)/single(1000),trim(arg_arg_voltage));Counter=Counter+uint16(1);
    |   else,Base=trim(arg_arg_voltage);end
    |   th=arg_arg_stick(4);if th>-.2 && th<.2,th=single(0);end
    |   Alt=min(max(single(double(Alt)+double(th)*.001),single(.05)),single(1.8));
    |   if arg_arg_rangeFlag>RangeOld || arg_arg_rangeFlag==20,Base=Base-single(.02);RangeOld=arg_arg_rangeFlag;end
    |   arg_arg_raw=single(double(Base)*3.7);
    |  else
    |   arg_arg_manual=true;th=min(max(arg_arg_stick(4),single(0)),single(1));
    |   if th>-.2 && th<.2,th=single(0);end
    |   arg_arg_raw=single((.00413+double(single(3.3)*th-single(5.44)*th*th+single(3.13)*th*th*th))*3.7);
    |  end
    | elseif arg_branch==5
    |  AltFlag=false;
    |  if ~Landing,Landing=true;History(:)=arg_arg_height;Base=trim(arg_arg_voltage);end
    |  if History(10)>=arg_arg_height,Base=single(double(Base)*.9999);end
    |  if arg_arg_height<.15,Base=single(double(Base)*.999);end
    |  if arg_arg_height<.1,Landing=false;end
    |  for j=2:10,History(j)=History(j-1);end
    |  History(1)=arg_arg_height;
    | end
    | arg_arg_alt=Alt;arg_arg_base=Base;arg_arg_counter=Counter;arg_arg_auto=AltFlag;arg_arg_controlMode=single(ControlMode);
    | end
    | function y=trim(v),y=-single(.2448)*v+single(1.5892);end

== stateflow chart StampFly_StudentBlocks/FlightSequence/FinalizeFlightMode ==
  state Calculate
    en: [mode]=stepFn(branch,preMode,height,flipStart,flipDone,overG);
    du: [mode]=stepFn(branch,preMode,height,flipStart,flipDone,overG);
  (default) -> Calculate
  data: arg_branch function_input; arg_preMode function_input; arg_height function_input; arg_flipStart function_input; arg_flipDone function_input; arg_overG function_input; arg_mode function_output; branch input uint8; preMode input uint8; height input single; flipStart input boolean; flipDone input boolean; overG input uint8; mode output uint8
  function arg_mode=stepFn(arg_branch,arg_preMode,arg_height,arg_flipStart,arg_flipDone,arg_overG):
    | function arg_mode=stepFn(arg_branch,arg_preMode,arg_height,arg_flipStart,arg_flipDone,arg_overG)
    | % loop分岐の途中で変わるMode。get_commandは分岐途中でもFlipに変更できる。
    | %#codegen
    | arg_mode=arg_preMode;
    | if arg_branch==5 && arg_height<.1,arg_mode=uint8(3);end
    | if arg_flipStart && (arg_branch==2 || arg_branch==6),arg_mode=uint8(6);end
    | if arg_branch==6 && arg_flipDone,arg_mode=uint8(2);end
    | if (arg_branch==2 || arg_branch==5 || arg_branch==6) && arg_overG==1,arg_mode=uint8(3);end
    | end

== stateflow chart StampFly_StudentBlocks/Estimation/IMUBiasCalibration ==
  note: 800周期の平均校正：ジャイロXYZと加速度Zのオフセットを平均します。400 Hzなので公称2秒です。
  state Calculate
    en: [offset,count]=stepFn(a,g,mode);
    du: [offset,count]=stepFn(a,g,mode);
  (default) -> Calculate
  data: a function_input; g function_input; mode function_input; offset function_output; count function_output; a input single; g input single; mode input uint8; offset output single; count output uint16
  function [offset,count]=stepFn(a,g,mode):
    | function [offset,count]=stepFn(a,g,mode)
    | % 日本語の説明はブロック注釈とDescriptionを参照。
    | %#codegen
    | persistent Offset Count;
    | if isempty(Offset)
    | Offset=zeros(4,1,'single');
    | Count=uint16(0);
    | end
    |             if mode==0,Offset(:)=single(0);Count=uint16(0);
    |             elseif mode==1 && Count<uint16(800)
    |                 n=single(Count);Offset=(n*Offset+[g;a(3)])/(n+single(1));Count=Count+uint16(1);
    |             end
    |             offset=Offset;count=Count;
    | end

== stateflow chart StampFly_StudentBlocks/FlightSequence/OfficialTakeoffHover400/OfficialFlightSupervisor ==
  note: 公式の状態監督：INIT=0 → AVERAGE=1 → PARKING=3 → FLIGHT=2。ボタン・通信喪失・センサー状態に応じて LANDING=5 へ遷移。押下・解放の判定順を公式と一致させる。
  state Calculate
    en: [branch,mode,ahrsReset,parkingReset,connected]=stepFn(previousMode,button,newPacket,flags,ahrsFlag);
    du: [branch,mode,ahrsReset,parkingReset,connected]=stepFn(previousMode,button,newPacket,flags,ahrsFlag);
  (default) -> Calculate
  data: arg_previousMode function_input; arg_button function_input; arg_newPacket function_input; arg_flags function_input; arg_ahrsFlag function_input; arg_branch function_output; arg_mode function_output; arg_ahrsReset function_output; arg_parkingReset function_output; arg_connected function_output; previousMode input uint8; button input uint8; newPacket input uint8; flags input uint8; ahrsFlag input uint8; branch output uint8; mode output uint8; ahrsReset output boolean; parkingReset output boolean; connected output uint8
  function [arg_branch,arg_mode,arg_ahrsReset,arg_parkingReset,arg_connected]=stepFn(arg_previousMode,arg_button,arg_newPacket,arg_flags,arg_ahrsFlag):
    | function [arg_branch,arg_mode,arg_ahrsReset,arg_parkingReset,arg_connected]=stepFn(arg_previousMode,arg_button,arg_newPacket,arg_flags,arg_ahrsFlag)
    | % 公式loop_400Hzの分岐開始時。遷移後も現在の分岐を最後まで実行する。
    | %#codegen
    | persistent calibration buttonCounter buttonState chatter lastAHRS connectionCounter;
    | if isempty(calibration)
    |  calibration=uint16(0);buttonCounter=int8(0);buttonState=uint8(0);
    |  chatter=uint8(0);lastAHRS=uint8(0);connectionCounter=uint16(0);
    | end
    | arg_branch=arg_previousMode;arg_mode=arg_branch;arg_ahrsReset=false;arg_parkingReset=arg_branch==3;
    | if arg_newPacket~=0,connectionCounter=uint16(0);end
    | arg_connected=uint8(connectionCounter<uint16(40));
    | if arg_branch==0,arg_mode=uint8(1);
    | elseif arg_branch==1
    |  if calibration<uint16(800),calibration=calibration+uint16(1);else,arg_mode=uint8(3);end
    | else
    |  if arg_button==1
    |   buttonCounter=buttonCounter+int8(1);
    |   if buttonCounter>int8(10),buttonCounter=int8(10);buttonState=uint8(1);end
    |  else
    |   buttonCounter=buttonCounter-int8(1);
    |   if buttonCounter<int8(-10),buttonCounter=int8(-10);buttonState=uint8(0);end
    |  end
    |  event=false;
    |  if chatter==0
    |   if buttonState==1,chatter=uint8(1);end
    |  elseif buttonState==0
    |   chatter=chatter+uint8(1);
    |   if chatter>uint8(40),chatter=uint8(0);event=true;end
    |  end
    |  if arg_branch==3
    |   if event,arg_mode=uint8(2);arg_ahrsReset=true;end
    |   if arg_ahrsFlag~=lastAHRS
    |    if arg_ahrsFlag==1,arg_ahrsReset=true;end
    |    lastAHRS=arg_ahrsFlag;
    |   end
    |  elseif arg_branch==2 || arg_branch==6
    |   connectionCounter=uint16(mod(double(connectionCounter)+1,65536));
    |   arg_connected=uint8(connectionCounter<uint16(40));
    |   if event,arg_mode=uint8(5);end
    |   if arg_connected==0,arg_mode=uint8(5);end
    |   if arg_flags(1)==1,arg_mode=uint8(3);end
    |   if arg_branch==2 && arg_mode~=arg_branch,arg_ahrsReset=true;end
    |  elseif arg_branch==5
    |   if event,arg_mode=uint8(3);end
    |  end
    | end
    | end

== stateflow chart StampFly_StudentBlocks/FlightSequence/OfficialTakeoffHover400/OfficialFlipSequence ==
  note: 公式 Flip：ボタンで開始し、推力・Roll角速度を段階的に切り替える。完了・中断時の保持値と推定器のリセットを公式の順に出力。USBベンチでは実モーター出力ゼロ。
  state Calculate
    en: [start,done,phase,thrust,rollRate,angleReset,ahrsReset,normalControl]=stepFn(button,branch,voltage,previousReset,lastRate);
    du: [start,done,phase,thrust,rollRate,angleReset,ahrsReset,normalControl]=stepFn(button,branch,voltage,previousReset,lastRate);
  (default) -> Calculate
  data: arg_arg_button function_input; arg_arg_branch function_input; arg_arg_voltage function_input; arg_arg_previousReset function_input; arg_arg_lastRate function_input; arg_arg_start function_output; arg_arg_done function_output; arg_arg_phase function_output; arg_arg_thrust function_output; arg_arg_rollRate function_output; arg_arg_angleReset function_output; arg_arg_ahrsReset function_output; arg_arg_normalControl function_output; button input uint8; branch input uint8; voltage input single; previousReset input boolean; lastRate input single; start output boolean; done output boolean; phase output uint8; thrust output single; rollRate output single; angleReset output boolean; ahrsReset output boolean; normalControl output boolean
  function [arg_arg_start,arg_arg_done,arg_arg_phase,arg_arg_thrust,arg_arg_rollRate,arg_arg_angleReset,arg_arg_ahrsReset,arg_arg_normalControl]=stepFn(arg_arg_button,arg_arg_branch,arg_arg_voltage,arg_arg_previousReset,arg_arg_lastRate):
    | function [arg_arg_start,arg_arg_done,arg_arg_phase,arg_arg_thrust,arg_arg_rollRate,arg_arg_angleReset,arg_arg_ahrsReset,arg_arg_normalControl]=stepFn(arg_arg_button,arg_arg_branch,arg_arg_voltage,arg_arg_previousReset,arg_arg_lastRate)
    | % 公式 flip(): 180 + 40*4 + 10 + 190 tick。制御は別のPIDブロック。
    | %#codegen
    | persistent counter buttonCount rate didReset;
    | if isempty(counter),counter=uint16(0);buttonCount=uint8(0);rate=single(0);didReset=false;end
    | arg_arg_start=false;arg_arg_done=false;arg_arg_phase=uint8(0);arg_arg_thrust=single(0);arg_arg_rollRate=single(0);arg_arg_angleReset=false;arg_arg_ahrsReset=false;arg_arg_normalControl=true;
    | if arg_arg_branch==3 || arg_arg_previousReset,counter=uint16(0);rate=single(0);didReset=false;end
    | if arg_arg_branch==6
    |  rate=arg_arg_lastRate(1);
    |  T=single(double(-single(.2448)*arg_arg_voltage+single(1.5892))*3.7);
    |  flipTime=single(.4);flipStep=uint16(fix(flipTime/single(.0025)));quarter=idivide(flipStep,uint16(4));
    |  domega=single(double(single(.00217))*8*pi/double(flipTime)/double(flipTime));
    |  if counter<180
    |   arg_arg_phase=uint8(1);arg_arg_normalControl=false;
    |   if arg_arg_voltage>3.8,arg_arg_thrust=single(double(T)+.17*3.7);else,arg_arg_thrust=single(double(T)+.15*3.7);end
    |  elseif counter<180+quarter
    |   arg_arg_phase=uint8(2);arg_arg_normalControl=false;arg_arg_thrust=T*single(.3);rate=rate+domega;
    |  elseif counter<180+2*quarter
    |   arg_arg_phase=uint8(3);arg_arg_normalControl=false;arg_arg_thrust=T*single(.15);rate=rate+domega;
    |  elseif counter<180+3*quarter
    |   arg_arg_phase=uint8(4);arg_arg_normalControl=false;arg_arg_thrust=T*single(.15);rate=rate-domega;
    |  elseif counter<180+flipStep
    |   arg_arg_phase=uint8(5);arg_arg_normalControl=false;arg_arg_thrust=T;rate=rate-domega;
    |  elseif counter<190+flipStep
    |   arg_arg_phase=uint8(6);arg_arg_normalControl=false;arg_arg_thrust=single(double(T)+double(single(.18))*3.7);rate=single(0);arg_arg_angleReset=true;
    |   if ~didReset,arg_arg_ahrsReset=true;didReset=true;end
    |  elseif counter<380+flipStep,arg_arg_normalControl=true;
    |  else,arg_arg_done=true;arg_arg_normalControl=false;counter=uint16(0);didReset=false;
    |  end
    |  arg_arg_rollRate=rate;if ~arg_arg_done,counter=counter+uint16(1);end
    | end
    | if arg_arg_branch==2 || (arg_arg_branch==6 && arg_arg_normalControl)
    |  if arg_arg_button==1
    |   buttonCount=buttonCount+uint8(1);
    |   if buttonCount>uint8(10),buttonCount=uint8(0);arg_arg_start=true;end
    |  else,buttonCount=uint8(0);end
    | end
    | end
